simulink model "Drone_swarm_control"  (R2025a)
settings: Solver=FixedStepAuto  StartTime=0.0  StopTime=180  FixedStep=0.001  RelTol=1e-3
InitFcn:
  | %% Simulation parameters and waypoint trajectory
  | % Initial drone positions.
  | init_0=[0;0;0];
  | d_s=4;
  | init_1=init_0+d_s*[-1.1;0.1;0];
  | init_2=init_0+d_s*[0.3;-1.5;0];
  | init_3=init_0+d_s*[1.6;0.4;0];
  | init_4=init_0+d_s*[0.2;1.8;0];
  | 
  | % Initial battery energy in Wh.
  | E_0=77;
  | gain_2=1;
  | 
  | % PID controller gains.
  | PID_p=20;
  | PID_i=50;
  | PID_d=0;
  | 
  | % Router queues and background traffic.
  | router_buffer=160;
  | router_bandwith=300;
  | router_init_queue=[20,0,0,0,0];
  | traffic_mean=20;
  | traffic_variance=1;
  | 
  | % Communication-rate parameters.
  | F_max=2;
  | F_min=0.5;
  | F_H=(F_max+F_min)/3;
  | P_nc=(1-(F_H-F_min)/F_max);
  | 
  | 
  | % Desired formation offsets.
  | init_f_0=[0;0;0];
  | d_f=10;
  | init_f_1=init_0+d_f*[-1;0;0];
  | init_f_2=init_0+d_f*[0;-1;0];
  | init_f_3=init_0+d_f*[1;0;0];
  | init_f_4=init_0+d_f*[0;1;0];
  | 
  | 
  | % Waypoint mission with a fixed cruise altitude.
  | quota_fissa = -20;
  | 
  | waypoints = [
  |       0   0   0   0;
  |      75   0   quota_fissa   0;
  |     150   0   quota_fissa   0;
  |     225   0   quota_fissa   0;
  |     300   0   quota_fissa   0;
  |     300   0   quota_fissa   0;
  |     225  75   quota_fissa   0;
  |     150 150   quota_fissa   0;
  |      75 225   quota_fissa   0;
  |       0 300   quota_fissa   0;
  |       0 300   quota_fissa   0;
  |      75 300   quota_fissa   0;
  |     150 300   quota_fissa   0;
  |     225 300   quota_fissa   0;
  |     300 300   quota_fissa   0;
  | ... (+79 lines)
undefined symbols (not defined in the file): A_diacenza, DiscIntNeverNeededParam, L
libraries: dspsigops x10, robotcorelib x5, slpidlib x5, dspstat3 x5, simulink x1, uavutilslib x1
(part 4 of 4)

== matlab function Drone_swarm_control/Subsystem1/Subsystem_1/Inner-loop control/Inner-loop control ==
  data: Rb_des output size=[3,3]; omega_bb_des output size=3; tau output size=3; zb_des input size=3; Rb input size=[3,3]; dot_Rb_des input size=[3,3]; omega_bb input size=3; dot_omega_bb_des input size=3; xb_des input size=3; Ib parameter size=[3,3]; err_R output size=3; err_W output size=3
function [Rb_des,omega_bb_des,tau,err_R,err_W] = fcn(zb_des,Rb,dot_Rb_des,omega_bb,dot_omega_bb_des,xb_des,Ib)
% Geometric attitude control from rotation and angular-velocity errors.


k_rx = 50;
k_ry = 50;
k_rz = 50;

k_wx = 50;
k_wy = 50;
k_wz = 50;

K_r = diag([k_rx, k_ry, k_rz]);
K_w = diag([k_wx, k_wy, k_wz]);


% Construct the desired rotation matrix from the requested body axes.
yb_des = (skew(zb_des)*xb_des)/norm(skew(zb_des)*xb_des);

Rb_des = [skew(yb_des)*zb_des, yb_des, zb_des];

omega_bb_des = wedge(Rb_des&apos;*dot_Rb_des);

err_R = 0.5*wedge(Rb_des&apos;*Rb - Rb&apos;*Rb_des);

err_W = omega_bb - Rb&apos;*Rb_des*omega_bb_des;

% Combine attitude feedback with rigid-body compensation.
tau = -K_r*err_R - K_w*err_W + skew(omega_bb)*Ib*omega_bb - Ib*(skew(omega_bb)*Rb&apos;*Rb_des*omega_bb_des-Rb&apos;*Rb_des*dot_omega_bb_des); 

end

function S = skew(v)
% Matrix representation of the cross product.
if(numel(v)~= 1)
S= [0 -v(3) v(2); 
    v(3) 0 -v(1);
    -v(2) v(1) 0];
else
S= zeros(3);
end
end

function v = wedge(S)
% Extract the vector associated with a skew-symmetric matrix.
v1 = S(3,2);
v2 = S(1,3);
v3 = S(2,1);
v = [v1 v2 v3]&apos;;
end

== matlab function Drone_swarm_control/Subsystem5/MATLAB Function ==
  data: vettore input; output output; waypoints input
function output = confrontaDistanza(vettore, waypoints)
% Flag when the position is within the waypoint-distance threshold.
    output = 0;
    matrice = waypoints(:, 1:3);
    for i = 1:size(matrice, 1)
        distanza = norm(vettore - matrice(i, :));
        if distanza < 0.65
            output = 1;
            break;
        end
    end
end

== matlab function Drone_swarm_control/Subsystem1/Subsystem_1/Outer-loop control ==
  data: position input size=3; uT output size=1; linear_vel input size=3; Rb input size=[3,3]; zb_des output size=3; mass parameter size=1; position_des input size=3; vel_linear_des input size=3; acc_linear_des input size=3; err_p output size=3; dot_err_p output size=3
function [uT, zb_des, err_p, dot_err_p] = fcn(position, linear_vel, Rb, mass, ...
    position_des, vel_linear_des, acc_linear_des)
% Outer-loop position control: compute thrust and the desired body z-axis.


k_px = 10;
k_py = 10;
k_pz = 20;

k_vx = 10;
k_vy = 10;
k_vz = 20;

K_p = diag([k_px, k_py, k_pz]);
K_v = diag([k_vx, k_vy, k_vz]);


g = 9.81;

e_3 = [0 0 1]&apos;;

err_p = position - position_des;

dot_err_p = linear_vel - vel_linear_des;

% Normalize the commanded force to obtain the desired thrust direction.
zb_des = -(-K_p*err_p-K_v*dot_err_p-mass*g*e_3+mass*acc_linear_des)/norm(-K_p*err_p-K_v*dot_err_p-mass*g*e_3+mass*acc_linear_des);

uT = -(-K_p*err_p-K_v*dot_err_p-mass*g*e_3+mass*acc_linear_des)&apos;*Rb*e_3;

== matlab function Drone_swarm_control/Subsystem1/Subsystem_1/Quadrotor dynamics/MATLAB Function1 ==
  data: Rb_temp input; Rb output
function Rb = fcn(Rb_temp)
% Project the integrated matrix back onto SO(3) using SVD.
    [U,S,V] = svd(Rb_temp);
    sigma = det(U*V&apos;);
    S_ = diag([1 1 sigma]);

    Rb = U*S_*V&apos;;
end

== matlab function Drone_swarm_control/Subsystem7/MATLAB Function4 ==
  data: v input; P output; a input; f input; E input; E_new output
function [P, E_new] = batteryDischargeXYZ(v, a, f, E)
% Estimate instantaneous power and update the remaining battery energy.

P_base = 130;
k_v = 0.69;
k_a = 10;
k_f = 0.001;

v_mag = norm(v);
a_mag = norm(a);

% Combine hovering, motion and packet-transmission power.
P = P_base + k_v * v_mag^2 + k_a * a_mag + k_f * f;

% Energy decrement using the existing 1 ms update step.
dE_dt = 0.001*(-P / 3600);

% Stop the decrement after battery depletion.
if E <= 0
    dE_dt = 0;
end

E_new=E+dE_dt;
end

== matlab function Drone_swarm_control/Subsystem1/Subsystem_2/Inner-loop control/Inner-loop control ==
  data: Rb_des output size=[3,3]; omega_bb_des output size=3; tau output size=3; zb_des input size=3; Rb input size=[3,3]; dot_Rb_des input size=[3,3]; omega_bb input size=3; dot_omega_bb_des input size=3; xb_des input size=3; Ib parameter size=[3,3]; err_R output size=3; err_W output size=3
function [Rb_des,omega_bb_des,tau,err_R,err_W] = fcn(zb_des,Rb,dot_Rb_des,omega_bb,dot_omega_bb_des,xb_des,Ib)
% Geometric attitude control from rotation and angular-velocity errors.


k_rx = 50;
k_ry = 50;
k_rz = 50;

k_wx = 50;
k_wy = 50;
k_wz = 50;

K_r = diag([k_rx, k_ry, k_rz]);
K_w = diag([k_wx, k_wy, k_wz]);


% Construct the desired rotation matrix from the requested body axes.
yb_des = (skew(zb_des)*xb_des)/norm(skew(zb_des)*xb_des);

Rb_des = [skew(yb_des)*zb_des, yb_des, zb_des];

omega_bb_des = wedge(Rb_des&apos;*dot_Rb_des);

err_R = 0.5*wedge(Rb_des&apos;*Rb - Rb&apos;*Rb_des);

err_W = omega_bb - Rb&apos;*Rb_des*omega_bb_des;

% Combine attitude feedback with rigid-body compensation.
tau = -K_r*err_R - K_w*err_W + skew(omega_bb)*Ib*omega_bb - Ib*(skew(omega_bb)*Rb&apos;*Rb_des*omega_bb_des-Rb&apos;*Rb_des*dot_omega_bb_des); 

end

function S = skew(v)
% Matrix representation of the cross product.
if(numel(v)~= 1)
S= [0 -v(3) v(2); 
    v(3) 0 -v(1);
    -v(2) v(1) 0];
else
S= zeros(3);
end
end

function v = wedge(S)
% Extract the vector associated with a skew-symmetric matrix.
v1 = S(3,2);
v2 = S(1,3);
v3 = S(2,1);
v = [v1 v2 v3]&apos;;
end

== matlab function Drone_swarm_control/Subsystem1/Subsystem_2/Outer-loop control ==
  data: position input size=3; uT output size=1; linear_vel input size=3; Rb input size=[3,3]; zb_des output size=3; mass parameter size=1; position_des input size=3; vel_linear_des input size=3; acc_linear_des input size=3; err_p output size=3; dot_err_p output size=3
function [uT, zb_des, err_p, dot_err_p] = fcn(position, linear_vel, Rb, mass, ...
    position_des, vel_linear_des, acc_linear_des)
% Outer-loop position control: compute thrust and the desired body z-axis.


k_px = 10;
k_py = 10;
k_pz = 20;

k_vx = 10;
k_vy = 10;
k_vz = 20;

K_p = diag([k_px, k_py, k_pz]);
K_v = diag([k_vx, k_vy, k_vz]);


g = 9.81;

e_3 = [0 0 1]&apos;;

err_p = position - position_des;

dot_err_p = linear_vel - vel_linear_des;

% Normalize the commanded force to obtain the desired thrust direction.
zb_des = -(-K_p*err_p-K_v*dot_err_p-mass*g*e_3+mass*acc_linear_des)/norm(-K_p*err_p-K_v*dot_err_p-mass*g*e_3+mass*acc_linear_des);

uT = -(-K_p*err_p-K_v*dot_err_p-mass*g*e_3+mass*acc_linear_des)&apos;*Rb*e_3;

== matlab function Drone_swarm_control/Subsystem1/Subsystem_2/Quadrotor dynamics/MATLAB Function1 ==
  data: Rb_temp input; Rb output
function Rb = fcn(Rb_temp)
% Project the integrated matrix back onto SO(3) using SVD.
    [U,S,V] = svd(Rb_temp);
    sigma = det(U*V&apos;);
    S_ = diag([1 1 sigma]);

    Rb = U*S_*V&apos;;
end

== matlab function Drone_swarm_control/Subsystem1/Subsystem_2/Quadrotor dynamics/UAV dynamics ==
  data: uT input size=1; tau_b input size=3; lin_acc output size=3; Rb input size=[3,3]; omega_bb input size=3; dot_Rb output size=[3,3]; ang_acc output size=3; mass parameter size=1; Ib parameter size=[3,3]
function [lin_acc, dot_Rb, ang_acc] = fcn(uT,tau_b,Rb,omega_bb,mass, Ib)
% Quadrotor translational and rotational rigid-body dynamics.

lin_acc = 9.81*[0 0 1]&apos;-(uT/mass)*Rb*[0 0 1]&apos;;
dot_Rb = Rb*skew(omega_bb);
ang_acc = inv(Ib)*(-skew(omega_bb)*Ib*omega_bb + tau_b);

end

function S = skew(v)
% Matrix representation of the cross product.
if(numel(v)~= 1)
S= [0 -v(3) v(2); 
    v(3) 0 -v(1);
    -v(2) v(1) 0];
else
S= zeros(3);
end
end

== matlab function Drone_swarm_control/Subsystem14/Subsystem/MATLAB Function3 ==
  data: x input; alpha input; vi output; A input; i input; delta_fault input
function vi = controllo_repulsivo(x, alpha, A, i,delta_fault)
% Repulsive velocity correction with an active-node mask.

    N = 5;
    dim = 3;
    
    v_out = zeros(N * dim, 1);
    
    % Position buffer for the stacked state.
    pos = zeros(dim, N);
    idx = (i - 1) * 9 + 1;
    pos(:, i) = x(idx : idx + 2);
    
    
    
    vi = zeros(dim, 1);
    pi = pos(:, i);
    for j = 2:N
        if A(i, j) == 1 && i ~= j && delta_fault(j)==1
            pj = pos(:, j);
            delta = pi - pj;
            norm_delta = norm(delta);
            if norm_delta > 0
                vi = vi + 200*alpha*delta * exp(-alpha*(norm_delta))-0.00054*norm_delta*delta;
            end
        end
    end
   
    
end

== matlab function Drone_swarm_control/Subsystem1/Subsystem_3/Inner-loop control/Inner-loop control ==
  data: Rb_des output size=[3,3]; omega_bb_des output size=3; tau output size=3; zb_des input size=3; Rb input size=[3,3]; dot_Rb_des input size=[3,3]; omega_bb input size=3; dot_omega_bb_des input size=3; xb_des input size=3; Ib parameter size=[3,3]; err_R output size=3; err_W output size=3
function [Rb_des,omega_bb_des,tau,err_R,err_W] = fcn(zb_des,Rb,dot_Rb_des,omega_bb,dot_omega_bb_des,xb_des,Ib)
% Geometric attitude control from rotation and angular-velocity errors.


k_rx = 50;
k_ry = 50;
k_rz = 50;

k_wx = 50;
k_wy = 50;
k_wz = 50;

K_r = diag([k_rx, k_ry, k_rz]);
K_w = diag([k_wx, k_wy, k_wz]);


% Construct the desired rotation matrix from the requested body axes.
yb_des = (skew(zb_des)*xb_des)/norm(skew(zb_des)*xb_des);

Rb_des = [skew(yb_des)*zb_des, yb_des, zb_des];

omega_bb_des = wedge(Rb_des&apos;*dot_Rb_des);

err_R = 0.5*wedge(Rb_des&apos;*Rb - Rb&apos;*Rb_des);

err_W = omega_bb - Rb&apos;*Rb_des*omega_bb_des;

% Combine attitude feedback with rigid-body compensation.
tau = -K_r*err_R - K_w*err_W + skew(omega_bb)*Ib*omega_bb - Ib*(skew(omega_bb)*Rb&apos;*Rb_des*omega_bb_des-Rb&apos;*Rb_des*dot_omega_bb_des); 

end

function S = skew(v)
% Matrix representation of the cross product.
if(numel(v)~= 1)
S= [0 -v(3) v(2); 
    v(3) 0 -v(1);
    -v(2) v(1) 0];
else
S= zeros(3);
end
end

function v = wedge(S)
% Extract the vector associated with a skew-symmetric matrix.
v1 = S(3,2);
v2 = S(1,3);
v3 = S(2,1);
v = [v1 v2 v3]&apos;;
end

== matlab function Drone_swarm_control/Subsystem1/Subsystem_3/Outer-loop control ==
  data: position input size=3; uT output size=1; linear_vel input size=3; Rb input size=[3,3]; zb_des output size=3; mass parameter size=1; position_des input size=3; vel_linear_des input size=3; acc_linear_des input size=3; err_p output size=3; dot_err_p output size=3
function [uT, zb_des, err_p, dot_err_p] = fcn(position, linear_vel, Rb, mass, ...
    position_des, vel_linear_des, acc_linear_des)
% Outer-loop position control: compute thrust and the desired body z-axis.


k_px = 10;
k_py = 10;
k_pz = 20;

k_vx = 10;
k_vy = 10;
k_vz = 20;

K_p = diag([k_px, k_py, k_pz]);
K_v = diag([k_vx, k_vy, k_vz]);


g = 9.81;

e_3 = [0 0 1]&apos;;

err_p = position - position_des;

dot_err_p = linear_vel - vel_linear_des;

% Normalize the commanded force to obtain the desired thrust direction.
zb_des = -(-K_p*err_p-K_v*dot_err_p-mass*g*e_3+mass*acc_linear_des)/norm(-K_p*err_p-K_v*dot_err_p-mass*g*e_3+mass*acc_linear_des);

uT = -(-K_p*err_p-K_v*dot_err_p-mass*g*e_3+mass*acc_linear_des)&apos;*Rb*e_3;

== matlab function Drone_swarm_control/Subsystem1/Subsystem_3/Quadrotor dynamics/MATLAB Function1 ==
  data: Rb_temp input; Rb output
function Rb = fcn(Rb_temp)
% Project the integrated matrix back onto SO(3) using SVD.
    [U,S,V] = svd(Rb_temp);
    sigma = det(U*V&apos;);
    S_ = diag([1 1 sigma]);

    Rb = U*S_*V&apos;;
end

== matlab function Drone_swarm_control/Subsystem1/Subsystem_3/Quadrotor dynamics/UAV dynamics ==
  data: uT input size=1; tau_b input size=3; lin_acc output size=3; Rb input size=[3,3]; omega_bb input size=3; dot_Rb output size=[3,3]; ang_acc output size=3; mass parameter size=1; Ib parameter size=[3,3]
function [lin_acc, dot_Rb, ang_acc] = fcn(uT,tau_b,Rb,omega_bb,mass, Ib)
% Quadrotor translational and rotational rigid-body dynamics.

lin_acc = 9.81*[0 0 1]&apos;-(uT/mass)*Rb*[0 0 1]&apos;;
dot_Rb = Rb*skew(omega_bb);
ang_acc = inv(Ib)*(-skew(omega_bb)*Ib*omega_bb + tau_b);

end

function S = skew(v)
% Matrix representation of the cross product.
if(numel(v)~= 1)
S= [0 -v(3) v(2); 
    v(3) 0 -v(1);
    -v(2) v(1) 0];
else
S= zeros(3);
end
end

== matlab function Drone_swarm_control/Subsystem1/Subsystem_4/Inner-loop control/Inner-loop control ==
  data: Rb_des output size=[3,3]; omega_bb_des output size=3; tau output size=3; zb_des input size=3; Rb input size=[3,3]; dot_Rb_des input size=[3,3]; omega_bb input size=3; dot_omega_bb_des input size=3; xb_des input size=3; Ib parameter size=[3,3]; err_R output size=3; err_W output size=3
function [Rb_des,omega_bb_des,tau,err_R,err_W] = fcn(zb_des,Rb,dot_Rb_des,omega_bb,dot_omega_bb_des,xb_des,Ib)
% Geometric attitude control from rotation and angular-velocity errors.


k_rx = 50;
k_ry = 50;
k_rz = 50;

k_wx = 50;
k_wy = 50;
k_wz = 50;

K_r = diag([k_rx, k_ry, k_rz]);
K_w = diag([k_wx, k_wy, k_wz]);


% Construct the desired rotation matrix from the requested body axes.
yb_des = (skew(zb_des)*xb_des)/norm(skew(zb_des)*xb_des);

Rb_des = [skew(yb_des)*zb_des, yb_des, zb_des];

omega_bb_des = wedge(Rb_des&apos;*dot_Rb_des);

err_R = 0.5*wedge(Rb_des&apos;*Rb - Rb&apos;*Rb_des);

err_W = omega_bb - Rb&apos;*Rb_des*omega_bb_des;

% Combine attitude feedback with rigid-body compensation.
tau = -K_r*err_R - K_w*err_W + skew(omega_bb)*Ib*omega_bb - Ib*(skew(omega_bb)*Rb&apos;*Rb_des*omega_bb_des-Rb&apos;*Rb_des*dot_omega_bb_des); 

end

function S = skew(v)
% Matrix representation of the cross product.
if(numel(v)~= 1)
S= [0 -v(3) v(2); 
    v(3) 0 -v(1);
    -v(2) v(1) 0];
else
S= zeros(3);
end
end

function v = wedge(S)
% Extract the vector associated with a skew-symmetric matrix.
v1 = S(3,2);
v2 = S(1,3);
v3 = S(2,1);
v = [v1 v2 v3]&apos;;
end

== matlab function Drone_swarm_control/Subsystem1/Subsystem_4/Outer-loop control ==
  data: position input size=3; uT output size=1; linear_vel input size=3; Rb input size=[3,3]; zb_des output size=3; mass parameter size=1; position_des input size=3; vel_linear_des input size=3; acc_linear_des input size=3; err_p output size=3; dot_err_p output size=3
function [uT, zb_des, err_p, dot_err_p] = fcn(position, linear_vel, Rb, mass, ...
    position_des, vel_linear_des, acc_linear_des)
% Outer-loop position control: compute thrust and the desired body z-axis.


k_px = 10;
k_py = 10;
k_pz = 20;

k_vx = 10;
k_vy = 10;
k_vz = 20;

K_p = diag([k_px, k_py, k_pz]);
K_v = diag([k_vx, k_vy, k_vz]);


g = 9.81;

e_3 = [0 0 1]&apos;;

err_p = position - position_des;

dot_err_p = linear_vel - vel_linear_des;

% Normalize the commanded force to obtain the desired thrust direction.
zb_des = -(-K_p*err_p-K_v*dot_err_p-mass*g*e_3+mass*acc_linear_des)/norm(-K_p*err_p-K_v*dot_err_p-mass*g*e_3+mass*acc_linear_des);

uT = -(-K_p*err_p-K_v*dot_err_p-mass*g*e_3+mass*acc_linear_des)&apos;*Rb*e_3;

== matlab function Drone_swarm_control/Subsystem1/Subsystem_4/Quadrotor dynamics/MATLAB Function1 ==
  data: Rb_temp input; Rb output
function Rb = fcn(Rb_temp)
% Project the integrated matrix back onto SO(3) using SVD.
    [U,S,V] = svd(Rb_temp);
    sigma = det(U*V&apos;);
    S_ = diag([1 1 sigma]);

    Rb = U*S_*V&apos;;
end

== matlab function Drone_swarm_control/Subsystem1/Subsystem_4/Quadrotor dynamics/UAV dynamics ==
  data: uT input size=1; tau_b input size=3; lin_acc output size=3; Rb input size=[3,3]; omega_bb input size=3; dot_Rb output size=[3,3]; ang_acc output size=3; mass parameter size=1; Ib parameter size=[3,3]
function [lin_acc, dot_Rb, ang_acc] = fcn(uT,tau_b,Rb,omega_bb,mass, Ib)
% Quadrotor translational and rotational rigid-body dynamics.

lin_acc = 9.81*[0 0 1]&apos;-(uT/mass)*Rb*[0 0 1]&apos;;
dot_Rb = Rb*skew(omega_bb);
ang_acc = inv(Ib)*(-skew(omega_bb)*Ib*omega_bb + tau_b);

end

function S = skew(v)
% Matrix representation of the cross product.
if(numel(v)~= 1)
S= [0 -v(3) v(2); 
    v(3) 0 -v(1);
    -v(2) v(1) 0];
else
S= zeros(3);
end
end

== matlab function Drone_swarm_control/Subsystem14/Subsystem5/MATLAB Function3 ==
  data: x input; alpha input; vi output; A input; i input; delta_fault input
function vi = controllo_repulsivo(x, alpha, A, i,delta_fault)
% Repulsive velocity correction with an active-node mask.

    N = 5;
    dim = 3;
    
    v_out = zeros(N * dim, 1);
    
    % Position buffer for the stacked state.
    pos = zeros(dim, N);
    idx = (i - 1) * 9 + 1;
    pos(:, i) = x(idx : idx + 2);
    
    
    
    vi = zeros(dim, 1);
    pi = pos(:, i);
    for j = 2:N
        if A(i, j) == 1 && i ~= j && delta_fault(j)==1
            pj = pos(:, j);
            delta = pi - pj;
            norm_delta = norm(delta);
            if norm_delta > 0
                vi = vi + 200*alpha*delta * exp(-alpha*(norm_delta))-0.00054*norm_delta*delta;
            end
        end
    end
   
    
end

== matlab function Drone_swarm_control/Subsystem1/Subsystem_5/Inner-loop control/Inner-loop control ==
  data: Rb_des output size=[3,3]; omega_bb_des output size=3; tau output size=3; zb_des input size=3; Rb input size=[3,3]; dot_Rb_des input size=[3,3]; omega_bb input size=3; dot_omega_bb_des input size=3; xb_des input size=3; Ib parameter size=[3,3]; err_R output size=3; err_W output size=3
function [Rb_des,omega_bb_des,tau,err_R,err_W] = fcn(zb_des,Rb,dot_Rb_des,omega_bb,dot_omega_bb_des,xb_des,Ib)
% Geometric attitude control from rotation and angular-velocity errors.


k_rx = 50;
k_ry = 50;
k_rz = 50;

k_wx = 50;
k_wy = 50;
k_wz = 50;

K_r = diag([k_rx, k_ry, k_rz]);
K_w = diag([k_wx, k_wy, k_wz]);


% Construct the desired rotation matrix from the requested body axes.
yb_des = (skew(zb_des)*xb_des)/norm(skew(zb_des)*xb_des);

Rb_des = [skew(yb_des)*zb_des, yb_des, zb_des];

omega_bb_des = wedge(Rb_des&apos;*dot_Rb_des);

err_R = 0.5*wedge(Rb_des&apos;*Rb - Rb&apos;*Rb_des);

err_W = omega_bb - Rb&apos;*Rb_des*omega_bb_des;

% Combine attitude feedback with rigid-body compensation.
tau = -K_r*err_R - K_w*err_W + skew(omega_bb)*Ib*omega_bb - Ib*(skew(omega_bb)*Rb&apos;*Rb_des*omega_bb_des-Rb&apos;*Rb_des*dot_omega_bb_des); 

end

function S = skew(v)
% Matrix representation of the cross product.
if(numel(v)~= 1)
S= [0 -v(3) v(2); 
    v(3) 0 -v(1);
    -v(2) v(1) 0];
else
S= zeros(3);
end
end

function v = wedge(S)
% Extract the vector associated with a skew-symmetric matrix.
v1 = S(3,2);
v2 = S(1,3);
v3 = S(2,1);
v = [v1 v2 v3]&apos;;
end

== matlab function Drone_swarm_control/Subsystem1/Subsystem_5/Outer-loop control ==
  data: position input size=3; uT output size=1; linear_vel input size=3; Rb input size=[3,3]; zb_des output size=3; mass parameter size=1; position_des input size=3; vel_linear_des input size=3; acc_linear_des input size=3; err_p output size=3; dot_err_p output size=3
function [uT, zb_des, err_p, dot_err_p] = fcn(position, linear_vel, Rb, mass, ...
    position_des, vel_linear_des, acc_linear_des)
% Outer-loop position control: compute thrust and the desired body z-axis.


k_px = 10;
k_py = 10;
k_pz = 20;

k_vx = 10;
k_vy = 10;
k_vz = 20;

K_p = diag([k_px, k_py, k_pz]);
K_v = diag([k_vx, k_vy, k_vz]);


g = 9.81;

e_3 = [0 0 1]&apos;;

err_p = position - position_des;

dot_err_p = linear_vel - vel_linear_des;

% Normalize the commanded force to obtain the desired thrust direction.
zb_des = -(-K_p*err_p-K_v*dot_err_p-mass*g*e_3+mass*acc_linear_des)/norm(-K_p*err_p-K_v*dot_err_p-mass*g*e_3+mass*acc_linear_des);

uT = -(-K_p*err_p-K_v*dot_err_p-mass*g*e_3+mass*acc_linear_des)&apos;*Rb*e_3;

== matlab function Drone_swarm_control/Subsystem1/Subsystem_5/Quadrotor dynamics/MATLAB Function1 ==
  data: Rb_temp input; Rb output
function Rb = fcn(Rb_temp)
% Project the integrated matrix back onto SO(3) using SVD.
    [U,S,V] = svd(Rb_temp);
    sigma = det(U*V&apos;);
    S_ = diag([1 1 sigma]);

    Rb = U*S_*V&apos;;
end

== matlab function Drone_swarm_control/Subsystem1/Subsystem_5/Quadrotor dynamics/UAV dynamics ==
  data: uT input size=1; tau_b input size=3; lin_acc output size=3; Rb input size=[3,3]; omega_bb input size=3; dot_Rb output size=[3,3]; ang_acc output size=3; mass parameter size=1; Ib parameter size=[3,3]
function [lin_acc, dot_Rb, ang_acc] = fcn(uT,tau_b,Rb,omega_bb,mass, Ib)
% Quadrotor translational and rotational rigid-body dynamics.

lin_acc = 9.81*[0 0 1]&apos;-(uT/mass)*Rb*[0 0 1]&apos;;
dot_Rb = Rb*skew(omega_bb);
ang_acc = inv(Ib)*(-skew(omega_bb)*Ib*omega_bb + tau_b);

end

function S = skew(v)
% Matrix representation of the cross product.
if(numel(v)~= 1)
S= [0 -v(3) v(2); 
    v(3) 0 -v(1);
    -v(2) v(1) 0];
else
S= zeros(3);
end
end

== matlab function Drone_swarm_control/Subsystem7/MATLAB Function5 ==
  data: v input; P output; a input; f input; E input; E_new output
function [P, E_new] = batteryDischargeXYZ(v, a, f, E)
% Estimate instantaneous power and update the remaining battery energy.

P_base = 130;
k_v = 0.69;
k_a = 10;
k_f = 0.001;

v_mag = norm(v);
a_mag = norm(a);

% Combine hovering, motion and packet-transmission power.
P = P_base + k_v * v_mag^2 + k_a * a_mag + k_f * f;

% Energy decrement using the existing 1 ms update step.
dE_dt = 0.001*(-P / 3600);

% Stop the decrement after battery depletion.
if E <= 0
    dE_dt = 0;
end

E_new=E+dE_dt;
end

== matlab function Drone_swarm_control/Subsystem14/Subsystem7/MATLAB Function3 ==
  data: x input; alpha input; vi output; A input; i input; delta_fault input
function vi = controllo_repulsivo(x, alpha, A, i,delta_fault)
% Repulsive velocity correction with an active-node mask.

    N = 5;
    dim = 3;
    
    v_out = zeros(N * dim, 1);
    
    % Position buffer for the stacked state.
    pos = zeros(dim, N);
    idx = (i - 1) * 9 + 1;
    pos(:, i) = x(idx : idx + 2);
    
    
    
    vi = zeros(dim, 1);
    pi = pos(:, i);
    for j = 2:N
        if A(i, j) == 1 && i ~= j && delta_fault(j)==1
            pj = pos(:, j);
            delta = pi - pj;
            norm_delta = norm(delta);
            if norm_delta > 0
                vi = vi + 200*alpha*delta * exp(-alpha*(norm_delta))-0.00054*norm_delta*delta;
            end
        end
    end
   
    
end

== matlab function Drone_swarm_control/Subsystem14/Subsystem8/MATLAB Function3 ==
  data: x input; alpha input; vi output; A input; i input; delta_fault input
function vi = controllo_repulsivo(x, alpha, A, i,delta_fault)
% Repulsive velocity correction with an active-node mask.

    N = 5;
    dim = 3;
    
    v_out = zeros(N * dim, 1);
    
    % Position buffer for the stacked state.
    pos = zeros(dim, N);
    idx = (i - 1) * 9 + 1;
    pos(:, i) = x(idx : idx + 2);
    
    
    
    vi = zeros(dim, 1);
    pi = pos(:, i);
    for j = 2:N
        if A(i, j) == 1 && i ~= j && delta_fault(j)==1
            pj = pos(:, j);
            delta = pi - pj;
            norm_delta = norm(delta);
            if norm_delta > 0
                vi = vi + 200*alpha*delta * exp(-alpha*(norm_delta))-0.00054*norm_delta*delta;
            end
        end
    end
   
    
end

== matlab function Drone_swarm_control/Subsystem14/Subsystem9/MATLAB Function3 ==
  data: x input; alpha input; vi output; A input; i input; delta_fault input
function vi = controllo_repulsivo(x, alpha, A, i,delta_fault)
% Repulsive velocity correction with an active-node mask.

    N = 5;
    dim = 3;
    
    v_out = zeros(N * dim, 1);
    
    % Position buffer for the stacked state.
    pos = zeros(dim, N);
    idx = (i - 1) * 9 + 1;
    pos(:, i) = x(idx : idx + 2);
    
    
    
    vi = zeros(dim, 1);
    pi = pos(:, i);
    for j = 2:N
        if A(i, j) == 1 && i ~= j && delta_fault(j)==1
            pj = pos(:, j);
            delta = pi - pj;
            norm_delta = norm(delta);
            if norm_delta > 0
                vi = vi + 200*alpha*delta * exp(-alpha*(norm_delta))-0.00054*norm_delta*delta;
            end
        end
    end
   
    
end

== matlab function Drone_swarm_control/trasmission/rate_min/MATLAB Function ==
  data: u input; y output
function y = fcn(u)
% Handle inactive channels before selecting a communication rate.


for i=1:5
    if u(i)==0
        u(i)=1000;
    end
end

% Reset the output when the minimum equals the fallback value.
if min(u)==1000
    u=zeros(5,1);
end
y = u;

end

== matlab function Drone_swarm_control/trasmission/rate_min/MATLAB Function1 ==
  data: u input; y output
function y = fcn(u)
% Handle inactive channels before selecting a communication rate.


for i=1:5
    if u(i)==0
        u(i)=1000;
    end
end

% Reset the output when the minimum equals the fallback value.
if min(u)==1000
    u=zeros(5,1);
end
y = u;

end
